simulink model "ASM_Traffic_MultiCore"  (R2026a)
settings: Solver=ode1  StartTime=SIM.tstart.v  StopTime=SIM.tend.v  FixedStep=SIM.StepSize.v
PostLoadFcn:
  | if any(exist('dsrtsu_mdlpostloadfcn', 'file') ~= 0), dsrtsu_mdlpostloadfcn('Execute', bdroot); end
  | try, asm_mdl_postloadfcn(bdroot, 'UpdateModel', 3600); catch, disp(lasterr); end,
InitFcn:
  | , if any(exist('rtifpga_mdlclblib', 'file') ~= 0), rtifpga_mdlclblib('Init', bdroot); end,
  | , if any(exist('dsmpb_private', 'file') ~= 0), dsmpb_private('dsmpb_mdlclblib', 'Init', bdroot); end,
model workspace (MAT data in the model file):
  asmReferencePath = [0 0.01 0.02 0.03 0.04 0.05 0.06 0.07 0.08 0.09 0.1 0.11 ... (350007 elements, 50001x7)]
  roadBounds : Simulink.Parameter (value not decoded)
  safetyAxes : Simulink.Parameter (value not decoded)
undefined symbols (not defined in the file): _to_, a0b2, ASM_BrakeHydraulics_DemoSystems, ASM_VehicleDynamics_DemoSystems, b98103fe8ad365046cd0, BrakeCircuit, controllerConfig, CPT, Crankshaft, DiscIntNeverNeededParam, dsmsi, FinalDriveAssembly, MDL, ModeSignals, mu, Pos_BrakePedal_Maneuver, rad, RefSignals, roadFamilyData, roadFamilyId, s_to_rpm, SIM, SoftECU, Suspension, Tire, Transmission
libraries: ASM_Traffic_lib x135, simulink x98, ASM_Utils_lib x77, ASM_VehicleDynamics_lib x70, ASM_Environment_lib x22, dsmpblib x20, dsmsilib x15, MDLD_Utils_lib x10, ASM_BrakeHydraulics_lib x3, sl_discontinuities x2
(part 24 of 65)

== system ASM_Traffic_MultiCore/Engine/Control/UserInterface/DISP_Control ==
  In : Inport
  Bus Selector2 : BusSelector  OutputSignals=Torque_Intervention.Enable_Trq_Request_Fast[0|1],Torque_Intervention.Enable_Trq_Request_Extern1[0|1],Torque_Intervention.Enable_Trq_Request_Extern2[0|1],Torque_Intervention.Enable_Trq_Request_Extern3[0|1],Torque_Intervention.Trq_Request_Fast[Nm],Torque_Intervention.Trq_Request_Extern1[Nm],Torque_Intervention.Trq_Request_Extern2[Nm],Torque_Intervention.Trq_Request_Extern3[Nm],Torque_Intervention.Pos_AccPedal_Request_Driver[%],Torque_Intervention.Pos_AccPedal_Request[%],EngineOperation.State_Engine[0|1|2|3|4],EngineOperation.Sw_Starter[0Off|1On]
  Enable_Trq_Request_Extern1[0|1] : Subsystem
      mask Display: disp('')
  Enable_Trq_Request_Extern2[0|1] : Subsystem
      mask Display: disp('')
  Enable_Trq_Request_Extern3[0|1] : Subsystem
      mask Display: disp('')
  Enable_Trq_Request_Fast[0|1] : Subsystem
      mask Display: disp('')
  Mux1 : Mux
  Mux2 : Mux  Inputs=2
  Mux3 : Mux
  Mux4 : Mux  Inputs=2
  Pos_AccPedal_Request[%] : Subsystem
      mask Display: disp('')
  Pos_AccPedal_Request_Driver[%] : Subsystem
      mask Display: disp('')
  SoftECU_Engine : Scope  NumInputPorts=4
      settings: TimeSpan=5  ActiveDisplayYMinimum=-42.03413  ActiveDisplayYMaximum=378.30719  DataLoggingMaxPoints=20000  DataLoggingDecimation=10
  State_Engine[0|1|2|3|4] : Subsystem
      mask Display: disp('')
  Sw_Starter[0|1] : Subsystem
      mask Display: disp('')
  Trq_Request_Extern1[Nm] : Subsystem
      mask Display: disp('')
  Trq_Request_Extern2[Nm] : Subsystem
      mask Display: disp('')
  Trq_Request_Extern3[Nm] : Subsystem
      mask Display: disp('')
  Trq_Request_Fast[Nm] : Subsystem
      mask Display: disp('')
  wires:
  In/1 -> Bus Selector2/1
  Bus Selector2/1 -> Enable_Trq_Request_Fast[0|1]/1(In1)  "<Enable_Trq_Request_Fast[0|1]>"
  Bus Selector2/2 -> Enable_Trq_Request_Extern1[0|1]/1(In1)  "<Enable_Trq_Request_Extern1[0|1]>"
  Bus Selector2/3 -> Enable_Trq_Request_Extern2[0|1]/1(In1)  "<Enable_Trq_Request_Extern2[0|1]>"
  Bus Selector2/4 -> Enable_Trq_Request_Extern3[0|1]/1(In1)  "<Enable_Trq_Request_Extern3[0|1]>"
  Bus Selector2/5 -> Trq_Request_Fast[Nm]/1(In1)  "<Trq_Request_Fast[Nm]>"
  Bus Selector2/6 -> Trq_Request_Extern1[Nm]/1(In1)  "<Trq_Request_Extern1[Nm]>"
  Bus Selector2/7 -> Trq_Request_Extern2[Nm]/1(In1)  "<Trq_Request_Extern2[Nm]>"
  Bus Selector2/8 -> Trq_Request_Extern3[Nm]/1(In1)  "<Trq_Request_Extern3[Nm]>"
  Bus Selector2/9 -> Pos_AccPedal_Request_Driver[%]/1(In1)  "<Pos_AccPedal_Request_Driver[%]>"
  Bus Selector2/10 -> Pos_AccPedal_Request[%]/1(In1)  "<Pos_AccPedal_Request[%]>"
  Bus Selector2/11 -> State_Engine[0|1|2|3|4]/1(In1)  "<State_Engine[0|1|2|3|4]>"
  Bus Selector2/12 -> Sw_Starter[0|1]/1(In1)  "<Sw_Starter[0Off|1On]>"
  Enable_Trq_Request_Fast[0|1]/1(Out1) -> Mux3/1
  Enable_Trq_Request_Extern1[0|1]/1(Out1) -> Mux3/2
  Enable_Trq_Request_Extern2[0|1]/1(Out1) -> Mux3/3
  Enable_Trq_Request_Extern3[0|1]/1(Out1) -> Mux3/4
  Trq_Request_Fast[Nm]/1(Out1) -> Mux1/1
  Trq_Request_Extern1[Nm]/1(Out1) -> Mux1/2
  Trq_Request_Extern2[Nm]/1(Out1) -> Mux1/3
  Trq_Request_Extern3[Nm]/1(Out1) -> Mux1/4
  Pos_AccPedal_Request_Driver[%]/1(Out1) -> Mux2/1
  Pos_AccPedal_Request[%]/1(Out1) -> Mux2/2
  Mux2/1 -> SoftECU_Engine/3
  State_Engine[0|1|2|3|4]/1(Out1) -> Mux4/1
  Sw_Starter[0|1]/1(Out1) -> Mux4/2
  Mux3/1 -> SoftECU_Engine/1
  Mux1/1 -> SoftECU_Engine/2
  Mux4/1 -> SoftECU_Engine/4

== system ASM_Traffic_MultiCore/Engine/Control/UserInterface/PAR_Control ==
  Termination : Constant  Value=0
  Out : Outport  VectorParamsAs1DForOutWhenUnconnected=off
  wires:
  Termination/1 -> Out/1

== system ASM_Traffic_MultiCore/Engine/Interface_In/ModelSignals/Enable_Trq_Decrease_Fast_ESP[0|1]_ ==
  In1 : Inport
  Gain : Gain  SaturateOnIntegerOverflow=on  OutDataTypeStr=Inherit: Same as input  ParamDataTypeStr=Inherit: Same as input
  Out1 : Outport  VectorParamsAs1DForOutWhenUnconnected=off
  wires:
  In1/1 -> Gain/1
  Gain/1 -> Out1/1

== system ASM_Traffic_MultiCore/Engine/Interface_In/ModelSignals/Enable_Trq_Increase_Fast_ESP[0|1]_ ==
  In1 : Inport
  Gain : Gain  SaturateOnIntegerOverflow=on  OutDataTypeStr=Inherit: Same as input  ParamDataTypeStr=Inherit: Same as input
  Out1 : Outport  VectorParamsAs1DForOutWhenUnconnected=off
  wires:
  In1/1 -> Gain/1
  Gain/1 -> Out1/1

== system ASM_Traffic_MultiCore/Engine/Interface_In/ModelSignals/Enable_Trq_Request_Extern1[0|1]_ ==
  In1 : Inport
  Gain : Gain  SaturateOnIntegerOverflow=on  OutDataTypeStr=Inherit: Same as input  ParamDataTypeStr=Inherit: Same as input
  Out1 : Outport  VectorParamsAs1DForOutWhenUnconnected=off
  wires:
  In1/1 -> Gain/1
  Gain/1 -> Out1/1

== system ASM_Traffic_MultiCore/Engine/Interface_In/ModelSignals/Enable_Trq_Request_Extern2[0|1]_ ==
  In1 : Inport
  Gain : Gain  SaturateOnIntegerOverflow=on  OutDataTypeStr=Inherit: Same as input  ParamDataTypeStr=Inherit: Same as input
  Out1 : Outport  VectorParamsAs1DForOutWhenUnconnected=off
  wires:
  In1/1 -> Gain/1
  Gain/1 -> Out1/1

== system ASM_Traffic_MultiCore/Engine/Interface_In/ModelSignals/Enable_n_Engine_Idle_Request[0|1]_ ==
  In1 : Inport
  Gain : Gain  SaturateOnIntegerOverflow=on  OutDataTypeStr=Inherit: Same as input  ParamDataTypeStr=Inherit: Same as input
  Out1 : Outport  VectorParamsAs1DForOutWhenUnconnected=off
  wires:
  Gain/1 -> Out1/1
  In1/1 -> Gain/1

== system ASM_Traffic_MultiCore/Engine/Interface_In/ModelSignals/Factor_Trq_Engine_Red[%]_ ==
  In1 : Inport
  Gain : Gain  SaturateOnIntegerOverflow=on  OutDataTypeStr=Inherit: Same as input  ParamDataTypeStr=Inherit: Same as input
  Out1 : Outport  VectorParamsAs1DForOutWhenUnconnected=off
  wires:
  In1/1 -> Gain/1
  Gain/1 -> Out1/1

== system ASM_Traffic_MultiCore/Engine/Interface_In/ModelSignals/Mode_StartButtonState[1Stim|2SoftECU]_ ==
  In1 : Inport
  Gain : Gain  SaturateOnIntegerOverflow=on  OutDataTypeStr=Inherit: Same as input  ParamDataTypeStr=Inherit: Same as input
  Out1 : Outport  VectorParamsAs1DForOutWhenUnconnected=off
  wires:
  In1/1 -> Gain/1
  Gain/1 -> Out1/1

== system ASM_Traffic_MultiCore/Engine/Interface_In/ModelSignals/Pos_AccPedal_Driver[%]_ ==
  In1 : Inport
  Gain : Gain  SaturateOnIntegerOverflow=on  OutDataTypeStr=Inherit: Same as input  ParamDataTypeStr=Inherit: Same as input
  Out1 : Outport  VectorParamsAs1DForOutWhenUnconnected=off
  wires:
  In1/1 -> Gain/1
  Gain/1 -> Out1/1

== system ASM_Traffic_MultiCore/Engine/Interface_In/ModelSignals/Reset_States[0|1]_ ==
  In1 : Inport
  Gain : Gain  SaturateOnIntegerOverflow=on  OutDataTypeStr=Inherit: Same as input  ParamDataTypeStr=Inherit: Same as input
  Out1 : Outport  VectorParamsAs1DForOutWhenUnconnected=off
  wires:
  In1/1 -> Gain/1
  Gain/1 -> Out1/1

== system ASM_Traffic_MultiCore/Engine/Interface_In/ModelSignals/State_StartButton[-1|0|1|2]_ ==
  In1 : Inport
  Gain : Gain  SaturateOnIntegerOverflow=on  OutDataTypeStr=Inherit: Same as input  ParamDataTypeStr=Inherit: Same as input
  Out1 : Outport  VectorParamsAs1DForOutWhenUnconnected=off
  wires:
  Gain/1 -> Out1/1
  In1/1 -> Gain/1

== system ASM_Traffic_MultiCore/Engine/Interface_In/ModelSignals/Sw_CrankShaft_Reset[0Disabled|1Enabled]_ ==
  In1 : Inport
  Gain : Gain  SaturateOnIntegerOverflow=on  OutDataTypeStr=Inherit: Same as input  ParamDataTypeStr=Inherit: Same as input
  Out1 : Outport  VectorParamsAs1DForOutWhenUnconnected=off
  wires:
  In1/1 -> Gain/1
  Gain/1 -> Out1/1

== system ASM_Traffic_MultiCore/Engine/Interface_In/ModelSignals/Sw_Ignition[0Off|1On]_ ==
  In1 : Inport
  Gain : Gain  SaturateOnIntegerOverflow=on  OutDataTypeStr=Inherit: Same as input  ParamDataTypeStr=Inherit: Same as input
  Out1 : Outport  VectorParamsAs1DForOutWhenUnconnected=off
  wires:
  In1/1 -> Gain/1
  Gain/1 -> Out1/1

== system ASM_Traffic_MultiCore/Engine/Interface_In/ModelSignals/Sw_ModelDeskPlottingInterface[0Disabled|1Enabled]_ ==
  In1 : Inport
  Gain : Gain
  Out1 : Outport
  wires:
  Gain/1 -> Out1/1
  In1/1 -> Gain/1

== system ASM_Traffic_MultiCore/Engine/Interface_In/ModelSignals/Sw_ModelPortBlocks[0Disabled|1Enabled]_ ==
  In1 : Inport
  Gain : Gain
  Out1 : Outport
  wires:
  Gain/1 -> Out1/1
  In1/1 -> Gain/1

== system ASM_Traffic_MultiCore/Engine/Interface_In/ModelSignals/Sw_StarterReq[0Off|1On]_ ==
  In1 : Inport
  Gain : Gain  SaturateOnIntegerOverflow=on  OutDataTypeStr=Inherit: Same as input  ParamDataTypeStr=Inherit: Same as input
  Out1 : Outport  VectorParamsAs1DForOutWhenUnconnected=off
  wires:
  In1/1 -> Gain/1
  Gain/1 -> Out1/1

== system ASM_Traffic_MultiCore/Engine/Interface_In/ModelSignals/Trq_Decrease_Request_Fast_ESP[Nm]_ ==
  In1 : Inport
  Gain : Gain  SaturateOnIntegerOverflow=on  OutDataTypeStr=Inherit: Same as input  ParamDataTypeStr=Inherit: Same as input
  Out1 : Outport  VectorParamsAs1DForOutWhenUnconnected=off
  wires:
  In1/1 -> Gain/1
  Gain/1 -> Out1/1

== system ASM_Traffic_MultiCore/Engine/Interface_In/ModelSignals/Trq_Increase_Request_Fast_ESP[Nm]_ ==
  In1 : Inport
  Gain : Gain  SaturateOnIntegerOverflow=on  OutDataTypeStr=Inherit: Same as input  ParamDataTypeStr=Inherit: Same as input
  Out1 : Outport  VectorParamsAs1DForOutWhenUnconnected=off
  wires:
  In1/1 -> Gain/1
  Gain/1 -> Out1/1

== system ASM_Traffic_MultiCore/Engine/Interface_In/ModelSignals/Trq_Request_Extern1[Nm]_ ==
  In1 : Inport
  Gain : Gain  SaturateOnIntegerOverflow=on  OutDataTypeStr=Inherit: Same as input  ParamDataTypeStr=Inherit: Same as input
  Out1 : Outport  VectorParamsAs1DForOutWhenUnconnected=off
  wires:
  In1/1 -> Gain/1
  Gain/1 -> Out1/1

== system ASM_Traffic_MultiCore/Engine/Interface_In/ModelSignals/Trq_Request_Extern2[Nm]_ ==
  In1 : Inport
  Gain : Gain  SaturateOnIntegerOverflow=on  OutDataTypeStr=Inherit: Same as input  ParamDataTypeStr=Inherit: Same as input
  Out1 : Outport  VectorParamsAs1DForOutWhenUnconnected=off
  wires:
  In1/1 -> Gain/1
  Gain/1 -> Out1/1

== system ASM_Traffic_MultiCore/Engine/Interface_In/ModelSignals/Trq_Request_ICE[Nm]_ ==
  In1 : Inport
  Gain : Gain  SaturateOnIntegerOverflow=on  OutDataTypeStr=Inherit: Same as input  ParamDataTypeStr=Inherit: Same as input
  Out1 : Outport  VectorParamsAs1DForOutWhenUnconnected=off
  wires:
  In1/1 -> Gain/1
  Gain/1 -> Out1/1

== system ASM_Traffic_MultiCore/Engine/Interface_In/ModelSignals/Vehicle_Topology[-2|-1|0|2]_ ==
  In1 : Inport
  Gain : Gain  SaturateOnIntegerOverflow=on  OutDataTypeStr=Inherit: Same as input  ParamDataTypeStr=Inherit: Same as input
  Out1 : Outport  VectorParamsAs1DForOutWhenUnconnected=off
  wires:
  In1/1 -> Gain/1
  Gain/1 -> Out1/1

== system ASM_Traffic_MultiCore/Engine/Interface_In/ModelSignals/n_Engine[rpm]_ ==
  In1 : Inport
  Gain : Gain  SaturateOnIntegerOverflow=on  OutDataTypeStr=Inherit: Same as input  ParamDataTypeStr=Inherit: Same as input
  Out1 : Outport  VectorParamsAs1DForOutWhenUnconnected=off
  wires:
  In1/1 -> Gain/1
  Gain/1 -> Out1/1

== system ASM_Traffic_MultiCore/Engine/Interface_In/ModelSignals/n_Engine_Idle_Request[rpm]_ ==
  In1 : Inport
  Gain : Gain  SaturateOnIntegerOverflow=on  OutDataTypeStr=Inherit: Same as input  ParamDataTypeStr=Inherit: Same as input
  Out1 : Outport  VectorParamsAs1DForOutWhenUnconnected=off
  wires:
  In1/1 -> Gain/1
  Gain/1 -> Out1/1

== system ASM_Traffic_MultiCore/Engine/Interface_In/ModelSignals/v_x_Vehicle[km|h]_ ==
  In1 : Inport
  Gain : Gain  SaturateOnIntegerOverflow=on  OutDataTypeStr=Inherit: Same as input  ParamDataTypeStr=Inherit: Same as input
  Out1 : Outport  VectorParamsAs1DForOutWhenUnconnected=off
  wires:
  In1/1 -> Gain/1
  Gain/1 -> Out1/1

== system ASM_Traffic_MultiCore/Engine/Interface_Out/Control_ModelSignals/CrankAngle_Cyl[aTDC]_ ==
  In1 : Inport
  DummyGain : Gain  SaturateOnIntegerOverflow=on  OutDataTypeStr=Inherit: Same as input  ParamDataTypeStr=Inherit: Same as input
  Out1 : Outport  VectorParamsAs1DForOutWhenUnconnected=off
  wires:
  DummyGain/1 -> Out1/1
  In1/1 -> DummyGain/1

== system ASM_Traffic_MultiCore/Engine/Interface_Out/Control_ModelSignals/Enable_Trq_Shift_Request[0|1]_ ==
  In1 : Inport
  Gain : Gain  SaturateOnIntegerOverflow=on  OutDataTypeStr=Inherit: Same as input  ParamDataTypeStr=Inherit: Same as input
  Out1 : Outport  VectorParamsAs1DForOutWhenUnconnected=off
  wires:
  Gain/1 -> Out1/1
  In1/1 -> Gain/1

== system ASM_Traffic_MultiCore/Engine/Interface_Out/Control_ModelSignals/EngOP_Num[]_ ==
  In1 : Inport
  DummyGain : Gain  SaturateOnIntegerOverflow=on  OutDataTypeStr=Inherit: Same as input  ParamDataTypeStr=Inherit: Same as input
  Out1 : Outport  VectorParamsAs1DForOutWhenUnconnected=off
  wires:
  In1/1 -> DummyGain/1
  DummyGain/1 -> Out1/1

== system ASM_Traffic_MultiCore/Engine/Interface_Out/Control_ModelSignals/Pos_AccPedal_Meas[%]_ ==
  In1 : Inport
  DummyGain : Gain  SaturateOnIntegerOverflow=on  OutDataTypeStr=Inherit: Same as input  ParamDataTypeStr=Inherit: Same as input
  Out1 : Outport  VectorParamsAs1DForOutWhenUnconnected=off
  wires:
  DummyGain/1 -> Out1/1
  In1/1 -> DummyGain/1

== system ASM_Traffic_MultiCore/Engine/Interface_Out/Control_ModelSignals/State_ICEngine[0|1|2|3|4]_ ==
  In1 : Inport
  Gain : Gain  SaturateOnIntegerOverflow=on  OutDataTypeStr=Inherit: Same as input  ParamDataTypeStr=Inherit: Same as input
  Out1 : Outport  VectorParamsAs1DForOutWhenUnconnected=off
  wires:
  In1/1 -> Gain/1
  Gain/1 -> Out1/1

== system ASM_Traffic_MultiCore/Engine/Interface_Out/Control_ModelSignals/State_StartStop[1Off|2NotReady|3Ready|4EngStopped]_ ==
  In1 : Inport
  Gain : Gain  SaturateOnIntegerOverflow=on  OutDataTypeStr=Inherit: Same as input  ParamDataTypeStr=Inherit: Same as input
  Out1 : Outport  VectorParamsAs1DForOutWhenUnconnected=off
  wires:
  In1/1 -> Gain/1
  Gain/1 -> Out1/1

== system ASM_Traffic_MultiCore/Engine/Interface_Out/Control_ModelSignals/Sw_Replace_Env[0|1]_ ==
  In1 : Inport
  DummyGain : Gain  SaturateOnIntegerOverflow=on  OutDataTypeStr=Inherit: Same as input  ParamDataTypeStr=Inherit: Same as input
  Out1 : Outport  VectorParamsAs1DForOutWhenUnconnected=off
  wires:
  DummyGain/1 -> Out1/1
  In1/1 -> DummyGain/1

== system ASM_Traffic_MultiCore/Engine/Interface_Out/Control_ModelSignals/Sw_Starter[0Off|1On]_ ==
  In1 : Inport
  Gain : Gain  SaturateOnIntegerOverflow=on  OutDataTypeStr=Inherit: Same as input  ParamDataTypeStr=Inherit: Same as input
  Out1 : Outport  VectorParamsAs1DForOutWhenUnconnected=off
  wires:
  In1/1 -> Gain/1
  Gain/1 -> Out1/1

== system ASM_Traffic_MultiCore/Engine/Interface_Out/Control_ModelSignals/T_Ambient[degC]_ ==
  In1 : Inport
  DummyGain : Gain  SaturateOnIntegerOverflow=on  OutDataTypeStr=Inherit: Same as input  ParamDataTypeStr=Inherit: Same as input
  Out1 : Outport  VectorParamsAs1DForOutWhenUnconnected=off
  wires:
  DummyGain/1 -> Out1/1
  In1/1 -> DummyGain/1

== system ASM_Traffic_MultiCore/Engine/Interface_Out/Control_ModelSignals/Trq_MeanEff_Engine_Meas[Nm]_ ==
  In1 : Inport
  DummyGain : Gain  SaturateOnIntegerOverflow=on  OutDataTypeStr=Inherit: Same as input  ParamDataTypeStr=Inherit: Same as input
  Out1 : Outport  VectorParamsAs1DForOutWhenUnconnected=off
  wires:
  DummyGain/1 -> Out1/1
  In1/1 -> DummyGain/1

== system ASM_Traffic_MultiCore/Engine/Interface_Out/Control_ModelSignals/Trq_Shift_Request[Nm]_ ==
  In1 : Inport
  Gain : Gain  SaturateOnIntegerOverflow=on  OutDataTypeStr=Inherit: Same as input  ParamDataTypeStr=Inherit: Same as input
  Out1 : Outport  VectorParamsAs1DForOutWhenUnconnected=off
  wires:
  In1/1 -> Gain/1
  Gain/1 -> Out1/1

== system ASM_Traffic_MultiCore/Engine/Interface_Out/Control_ModelSignals/n_Engine_Idle_Set[rpm]_ ==
  In1 : Inport
  Gain : Gain  SaturateOnIntegerOverflow=on  OutDataTypeStr=Inherit: Same as input  ParamDataTypeStr=Inherit: Same as input
  Out1 : Outport  VectorParamsAs1DForOutWhenUnconnected=off
  wires:
  In1/1 -> Gain/1
  Gain/1 -> Out1/1

== system ASM_Traffic_MultiCore/Engine/Interface_Out/Control_ModelSignals/n_Engine_Meas[rpm]_ ==
  In1 : Inport
  DummyGain : Gain  SaturateOnIntegerOverflow=on  OutDataTypeStr=Inherit: Same as input  ParamDataTypeStr=Inherit: Same as input
  Out1 : Outport  VectorParamsAs1DForOutWhenUnconnected=off
  wires:
  In1/1 -> DummyGain/1
  DummyGain/1 -> Out1/1

== system ASM_Traffic_MultiCore/Engine/Interface_Out/Control_ModelSignals/p_Ambient[Pa]_ ==
  In1 : Inport
  DummyGain : Gain  SaturateOnIntegerOverflow=on  OutDataTypeStr=Inherit: Same as input  ParamDataTypeStr=Inherit: Same as input
  Out1 : Outport  VectorParamsAs1DForOutWhenUnconnected=off
  wires:
  In1/1 -> DummyGain/1
  DummyGain/1 -> Out1/1

== system ASM_Traffic_MultiCore/Engine/Interface_Out/Plant_ModelSignals/T_Coolant_ICE[degC]_ ==
  In1 : Inport
  Gain : Gain  SaturateOnIntegerOverflow=on  OutDataTypeStr=Inherit: Same as input  ParamDataTypeStr=Inherit: Same as input
  Out1 : Outport  VectorParamsAs1DForOutWhenUnconnected=off
  wires:
  Gain/1 -> Out1/1
  In1/1 -> Gain/1

== system ASM_Traffic_MultiCore/Engine/Interface_Out/Plant_ModelSignals/Trq_Fric_Engine[Nm]_ ==
  In1 : Inport
  Gain : Gain  SaturateOnIntegerOverflow=on  OutDataTypeStr=Inherit: Same as input  ParamDataTypeStr=Inherit: Same as input
  Out1 : Outport  VectorParamsAs1DForOutWhenUnconnected=off
  wires:
  In1/1 -> Gain/1
  Gain/1 -> Out1/1

== system ASM_Traffic_MultiCore/Engine/Interface_Out/Plant_ModelSignals/Trq_MeanEff_Engine[Nm]_ ==
  In1 : Inport
  Gain : Gain  SaturateOnIntegerOverflow=on  OutDataTypeStr=Inherit: Same as input  ParamDataTypeStr=Inherit: Same as input
  Out1 : Outport  VectorParamsAs1DForOutWhenUnconnected=off
  wires:
  In1/1 -> Gain/1
  Gain/1 -> Out1/1

== system ASM_Traffic_MultiCore/Engine/Interface_Out/Plant_ModelSignals/Type_Engine[0Unkown|1Other|2Otto|3Diesel|4Electric]_ ==
  In1 : Inport
  DummyGain : Gain  SaturateOnIntegerOverflow=on  OutDataTypeStr=Inherit: Same as input  ParamDataTypeStr=Inherit: Same as input
  Out1 : Outport  VectorParamsAs1DForOutWhenUnconnected=off
  wires:
  In1/1 -> DummyGain/1
  DummyGain/1 -> Out1/1

== system ASM_Traffic_MultiCore/Engine/Plant/EngineBasic/ASMSignalCollector ==
  BusCreator : BusCreator  Inputs=2
  ASMSIgnalBus : Outport  VectorParamsAs1DForOutWhenUnconnected=off
  wires:
  [ASMBUS_FUEL_CONSUMPTION] -> BusCreator/2
  BusCreator/1 -> ASMSIgnalBus/1  "Plant"
  [ASMBUS_ENGINE] -> BusCreator/1

== system ASM_Traffic_MultiCore/Engine/Plant/UserInterface/ASMSignalBus_Plant ==
  In : Inport
  Terminator_1 : Terminator
  tag scope: ASMBUS_Engine_Plant=global
  wires:
  [ASMBUS_Engine_Plant] -> Terminator_1/1
  In/1 -> [ASMBUS_Engine_Plant]  "Plant"

== system ASM_Traffic_MultiCore/Engine/Plant/UserInterface/DISP_Plant ==
  note: Dummy blocks for ControlDesk layout.
      | Might be replaced when simulating virtual vehicles.
  Interface_In : Inport
  In : Inport  Port=2
  Bus Selector1 : BusSelector  OutputSignals=Engine.Trq_Eff_Engine[Nm],Engine.Trq_Fric_Engine[Nm],Engine.Trq_Ind_Engine[Nm]
  Bus Selector10 : BusSelector  OutputSignals=FuelConsumption.CO2_Emission.CO2_Emission[kg|h],FuelConsumption.CO2_Emission.CO2_Emission_Total[kg],FuelConsumption.Fuel_Consumption[l|h],FuelConsumption.Fuel_Consumption_Total[l],FuelConsumption.mdot_Fuel[g|h],FuelConsumption.b_e[g|kWh],FuelConsumption.Efficiency.eta_Eff_Engine[0_1],FuelConsumption.Efficiency.eta_Ind_Engine[0_1],FuelConsumption.Efficiency.eta_Mechanical_Engine[0_1]
  Bus Selector2 : BusSelector  OutputSignals=ExternalModel.v_x_Vehicle[km|h]
  CO2_Emission[kg|100km] : Subsystem
      mask Display: disp('')
  CO2_Emission[kg|100km]_ : Subsystem
  CO2_Emission[kg|h] : Subsystem
      mask Display: disp('')
  CO2_Emission_Total[kg] : Subsystem
      mask Display: disp('')
  CarbonEmission : Scope  NumInputPorts=3
      settings: TimeSpan=5  ActiveDisplayYMinimum=98.25  ActiveDisplayYMaximum=102.25  DataLoggingMaxPoints=20000  DataLoggingDecimation=10  DataLoggingVariableName=ScopeData3
  Efficiency : Scope  NumInputPorts=3
      settings: TimeSpan=5  ActiveDisplayYMinimum=-0.1  ActiveDisplayYMaximum=0.6  DataLoggingMaxPoints=20000  DataLoggingDecimation=10  DataLoggingVariableName=ScopeData4
  Engine : Scope  NumInputPorts=3
      settings: TimeSpan=5  ActiveDisplayYMinimum=-20  ActiveDisplayYMaximum=110  DataLoggingMaxPoints=20000  DataLoggingDecimation=10  DataLoggingVariableName=ScopeData5
  FuelConsumption : Scope  NumInputPorts=5
      settings: TimeSpan=5  ActiveDisplayYMinimum=2100  ActiveDisplayYMaximum=2300  DataLoggingMaxPoints=20000  DataLoggingDecimation=10  DataLoggingVariableName=ScopeData6
  FuelTank : Constant  Value=0.5
  FuelTank[0|1] : Subsystem
      mask Display: disp('')
  Fuel_Consumption[L|100km] : Subsystem
      mask Display: disp('')
  Fuel_Consumption[L|100km]_ : Subsystem
  Fuel_Consumption[l|h] : Subsystem
      mask Display: disp('')
  Fuel_Consumption_Total[l] : Subsystem
      mask Display: disp('')
  T_Water : Constant
  T_Water[degC] : Subsystem
      mask Display: disp('')
  Terminator : Terminator
  Terminator2 : Terminator
  Trq_Eff_Engine[Nm] : Subsystem
      mask Display: disp('')
  Trq_Fric_Engine[Nm] : Subsystem
      mask Display: disp('')
  Trq_Ind_Engine[Nm] : Subsystem
      mask Display: disp('')
  b_e[g|kWh] : Subsystem
      mask Display: disp('')
  eta_Eff_Engine[0_1] : Subsystem
      mask Display: disp('')
  eta_Ind_Engine[0_1] : Subsystem
      mask Display: disp('')
  eta_Mechanical_Engine[0_1] : Subsystem
      mask Display: disp('')
  mdot_Fuel[g|h] : Subsystem
      mask Display: disp('')
  wires:
  Bus Selector2/1 -> CO2_Emission[kg|100km]_/1(v_Vehicle[km|h]), Fuel_Consumption[L|100km]_/1(v_Vehicle[km|h])  "<v_x_Vehicle[km|h]>"
  Interface_In/1 -> Bus Selector2/1
  Bus Selector10/4 -> Fuel_Consumption_Total[l]/1(In1)  "<Fuel_Consumption_Total[l]>"
  T_Water[degC]/1(Out1) -> Terminator2/1
  FuelTank/1 -> FuelTank[0|1]/1(In1)
  Fuel_Consumption[L|100km]/1(Out1) -> FuelConsumption/1  "Fuel_Conumption[l|100km]"
  T_Water/1 -> T_Water[degC]/1(In1)
  FuelTank[0|1]/1(Out1) -> Terminator/1
  Trq_Ind_Engine[Nm]/1(Out1) -> Engine/3  "Trq_Ind_Engine[Nm]"
  Bus Selector1/1 -> Trq_Eff_Engine[Nm]/1(In1)  "<Trq_Eff_Engine[Nm]>"
  Fuel_Consumption[L|100km]_/1(Fuel_Consumption[L|100km]) -> Fuel_Consumption[L|100km]/1(In1)
  Bus Selector1/3 -> Trq_Ind_Engine[Nm]/1(In1)  "<Trq_Ind_Engine[Nm]>"
  Trq_Fric_Engine[Nm]/1(Out1) -> Engine/2  "Trq_Fric_Engine[Nm]"
  CO2_Emission_Total[kg]/1(Out1) -> CarbonEmission/3  "CO2_Emission_Total[kg]"
  Bus Selector10/3 -> Fuel_Consumption[l|h]/1(In1), Fuel_Consumption[L|100km]_/2(Fuel_Consumption[l|h])  "<Fuel_Consumption[l|h]>"
  Bus Selector1/2 -> Trq_Fric_Engine[Nm]/1(In1)  "<Trq_Fric_Engine[Nm]>"
  CO2_Emission[kg|100km]_/1(CO2_Emission[kg|100km]) -> CO2_Emission[kg|100km]/1(In1)
  eta_Eff_Engine[0_1]/1(Out1) -> Efficiency/1  "eta_Eff_Engine[0_1]"
  Bus Selector10/5 -> mdot_Fuel[g|h]/1(In1)  "<mdot_Fuel[g|h]>"
  Bus Selector10/1 -> CO2_Emission[kg|h]/1(In1), CO2_Emission[kg|100km]_/2(CO2_Emission[kg|h])  "<CO2_Emission[kg|h]>"
  Bus Selector10/6 -> b_e[g|kWh]/1(In1)  "<b_e[g|kWh]>"
  Bus Selector10/2 -> CO2_Emission_Total[kg]/1(In1)  "<CO2_Emission_Total[kg]>"
  Trq_Eff_Engine[Nm]/1(Out1) -> Engine/1  "Trq_Eff_Engine[Nm]"
  CO2_Emission[kg|h]/1(Out1) -> CarbonEmission/2  "CO2_Emission[kg|h]"
  Bus Selector10/7 -> eta_Eff_Engine[0_1]/1(In1)  "<eta_Eff_Engine[0_1]>"
  Fuel_Consumption_Total[l]/1(Out1) -> FuelConsumption/3  "Fuel_Consumption_Total[l]"
  Bus Selector10/9 -> eta_Mechanical_Engine[0_1]/1(In1)  "<eta_Mechanical_Engine[0_1]>"
  In/1 -> Bus Selector1/1, Bus Selector10/1
  Fuel_Consumption[l|h]/1(Out1) -> FuelConsumption/2  "Fuel_Consumption[l|h]"
  eta_Mechanical_Engine[0_1]/1(Out1) -> Efficiency/3  "eta_Mechanical_Engine[0_1]"
  Bus Selector10/8 -> eta_Ind_Engine[0_1]/1(In1)  "<eta_Ind_Engine[0_1]>"
  eta_Ind_Engine[0_1]/1(Out1) -> Efficiency/2  "eta_Ind_Engine[0_1]"
  CO2_Emission[kg|100km]/1(Out1) -> CarbonEmission/1  "CO2_Emission[kg|100km]"
  b_e[g|kWh]/1(Out1) -> FuelConsumption/5  "b_e[g|kWh]"
  mdot_Fuel[g|h]/1(Out1) -> FuelConsumption/4  "mdot_Fuel[g|h]"

== system ASM_Traffic_MultiCore/Engine/Plant/UserInterface/PAR_Plant ==
  Termination : Constant  Value=0
  Out : Outport  VectorParamsAs1DForOutWhenUnconnected=off
  wires:
  Termination/1 -> Out/1

== system ASM_Traffic_MultiCore/Engine/SignalInterface/ASMSignalInterface/signal_structure ==
  ASMSignalBus : Inport
  BusSelector_1 : BusSelector  OutputSignals=Control,Plant
  CO2_Emission : BusSelector  OutputSignals=CO2_Emission[kg|h],CO2_Emission_Total[kg]
  ContentID : Constant  Value=278498219
  Control : BusSelector  OutputSignals=ESP_Fast_Torque_Set,Shift_Torque_Set,Torque_Intervention,IdleSpeedControl,EngineOperation
  DataTypeConversion_2 : DataTypeConversion  OutDataTypeStr=double
  ESP_Fast_Torque_Set : BusSelector  OutputSignals=Sw_Engine_Dynamics_Fast[0|1],Enable_Trq_Request_Fast[0|1],Trq_Request_Fast[Nm]
  Efficiency : BusSelector  OutputSignals=eta_Eff_Engine[0_1],eta_Ind_Engine[0_1],eta_Mechanical_Engine[0_1]
  Engine : BusSelector  OutputSignals=TimeConst_Engine_Dynamics[s],Trq_Eff_Engine[Nm],Trq_Driver_Des[Nm],Trq_FullLoad_Engine[Nm],Trq_Fric_Engine[Nm],Trq_Ind_Engine[Nm],Trq_Driver_Ind_Des[Nm],Trq_Engine_Ind_Max[Nm]
  EngineOperation : BusSelector  OutputSignals=State_Engine[0|1|2|3|4],Sw_Starter[0Off|1On]
  FuelConsumption : BusSelector  OutputSignals=mdot_Fuel[g|h],b_e[g|kWh],Efficiency,CO2_Emission,Fuel_Consumption[l|h],Fuel_Consumption_Total[l]
  IdleSpeedControl : BusSelector  OutputSignals=n_Engine_Idle_Set[rpm],Pos_AccPedal_Ctrl[%]
  InfoBlock : Subsystem
      mask Display: fprintf('Structural changes of the signal bus require an update \nof the ''ASMSignalCollector'' block. \n\nTo start the update process double click the parent block.\n\n WARNING:\n During update this subsystem will be cleared completely')
  MDLD_DATA_CAPTURE : MDLD_Utils_lib/ModelDeskPlotInterface/DataCapture_Sfcn/MDLD_DATA_CAPTURE  inputPortWidth=41  measurementSignals=[0 0 0 0 0 0 0 0 0 0 0 0 0 0 0 0 0 0 0 0 0 0 0 0 0 0 0 0 0 0 0 0 0 0 0 0 0 0 0 0 0]  downsampling=1  samplingPeriod=SIM.StepSize.v  uuid=0  ASMProperties=struct('Name','mdld_data_capture','Version','1.0','Library','mdld_utils_lib')  startTriggerDelay=0  startTriggerLogic=0  startTriggerCount=0  startTriggerConditions=[0,0,0,0,0,0,0,0,0]  stopTriggerDelay=0  stopTriggerLogic=0  stopTriggerCount=0  stopTriggerConditions=[0,0,0,0,0,0,0,0,0]  ContentID_RefStruct=278498219
  Plant : BusSelector  OutputSignals=Engine,FuelConsumption
  Shift_Torque_Set : BusSelector  OutputSignals=Trq_Driver_Ind_Des[Nm],Trq_Ind_Set[Nm],Enable_Trq_Ind_Set[0|1]
  SignalFilter : Mux  Inputs=41
  SignalFilterGain : Gain
  Terminator : Terminator
  Torque_Intervention : BusSelector  OutputSignals=Pos_AccPedal_Request[%],Enable_Trq_Request_Fast[0|1],Enable_Trq_Request_Extern1[0|1],Enable_Trq_Request_Extern2[0|1],Enable_Trq_Request_Extern3[0|1],Trq_Request_Fast[Nm],Trq_Request_Extern1[Nm],Trq_Request_Extern2[Nm],Trq_Request_Extern3[Nm],Pos_AccPedal_Request_Fast[%],Pos_AccPedal_Request_Extern1[%],Pos_AccPedal_Request_Extern2[%],Pos_AccPedal_Request_Extern3[%],Pos_AccPedal_Request_Driver[%]
  wires:
  ASMSignalBus/1 -> BusSelector_1/1
  BusSelector_1/1 -> Control/1  "<Control>"
  Control/1 -> ESP_Fast_Torque_Set/1  "<ESP_Fast_Torque_Set>"
  Control/2 -> Shift_Torque_Set/1  "<Shift_Torque_Set>"
  Control/3 -> Torque_Intervention/1  "<Torque_Intervention>"
  Control/4 -> IdleSpeedControl/1  "<IdleSpeedControl>"
  Control/5 -> EngineOperation/1  "<EngineOperation>"
  BusSelector_1/2 -> Plant/1  "<Plant>"
  Plant/1 -> Engine/1  "<Engine>"
  Plant/2 -> FuelConsumption/1  "<FuelConsumption>"
  FuelConsumption/3 -> Efficiency/1  "<Efficiency>"
  FuelConsumption/4 -> CO2_Emission/1  "<CO2_Emission>"
  ContentID/1 -> Terminator/1
  ESP_Fast_Torque_Set/1 -> SignalFilter/1  "<Sw_Engine_Dynamics_Fast[0|1]>"
  ESP_Fast_Torque_Set/2 -> DataTypeConversion_2/1  "<Enable_Trq_Request_Fast[0|1]>"
  DataTypeConversion_2/1 -> SignalFilter/2
  ESP_Fast_Torque_Set/3 -> SignalFilter/3  "<Trq_Request_Fast[Nm]>"
  Shift_Torque_Set/1 -> SignalFilter/4  "<Trq_Driver_Ind_Des[Nm]>"
  Shift_Torque_Set/2 -> SignalFilter/5  "<Trq_Ind_Set[Nm]>"
  Shift_Torque_Set/3 -> SignalFilter/6  "<Enable_Trq_Ind_Set[0|1]>"
  Torque_Intervention/1 -> SignalFilter/7  "<Pos_AccPedal_Request[%]>"
  Torque_Intervention/2 -> SignalFilter/8  "<Enable_Trq_Request_Fast[0|1]>"
  Torque_Intervention/3 -> SignalFilter/9  "<Enable_Trq_Request_Extern1[0|1]>"
  Torque_Intervention/4 -> SignalFilter/10  "<Enable_Trq_Request_Extern2[0|1]>"
  Torque_Intervention/5 -> SignalFilter/11  "<Enable_Trq_Request_Extern3[0|1]>"
  Torque_Intervention/6 -> SignalFilter/12  "<Trq_Request_Fast[Nm]>"
  Torque_Intervention/7 -> SignalFilter/13  "<Trq_Request_Extern1[Nm]>"
  Torque_Intervention/8 -> SignalFilter/14  "<Trq_Request_Extern2[Nm]>"
  Torque_Intervention/9 -> SignalFilter/15  "<Trq_Request_Extern3[Nm]>"
  Torque_Intervention/10 -> SignalFilter/16  "<Pos_AccPedal_Request_Fast[%]>"
  Torque_Intervention/11 -> SignalFilter/17  "<Pos_AccPedal_Request_Extern1[%]>"
  Torque_Intervention/12 -> SignalFilter/18  "<Pos_AccPedal_Request_Extern2[%]>"
  Torque_Intervention/13 -> SignalFilter/19  "<Pos_AccPedal_Request_Extern3[%]>"
  Torque_Intervention/14 -> SignalFilter/20  "<Pos_AccPedal_Request_Driver[%]>"
  IdleSpeedControl/1 -> SignalFilter/21  "<n_Engine_Idle_Set[rpm]>"
  IdleSpeedControl/2 -> SignalFilter/22  "<Pos_AccPedal_Ctrl[%]>"
  EngineOperation/1 -> SignalFilter/23  "<State_Engine[0|1|2|3|4]>"
  EngineOperation/2 -> SignalFilter/24  "<Sw_Starter[0Off|1On]>"
  Engine/1 -> SignalFilter/25  "<TimeConst_Engine_Dynamics[s]>"
  Engine/2 -> SignalFilter/26  "<Trq_Eff_Engine[Nm]>"
  Engine/3 -> SignalFilter/27  "<Trq_Driver_Des[Nm]>"
  Engine/4 -> SignalFilter/28  "<Trq_FullLoad_Engine[Nm]>"
  Engine/5 -> SignalFilter/29  "<Trq_Fric_Engine[Nm]>"
  Engine/6 -> SignalFilter/30  "<Trq_Ind_Engine[Nm]>"
  Engine/7 -> SignalFilter/31  "<Trq_Driver_Ind_Des[Nm]>"
  Engine/8 -> SignalFilter/32  "<Trq_Engine_Ind_Max[Nm]>"
  FuelConsumption/1 -> SignalFilter/33  "<mdot_Fuel[g|h]>"
  FuelConsumption/2 -> SignalFilter/34  "<b_e[g|kWh]>"
  Efficiency/1 -> SignalFilter/35  "<eta_Eff_Engine[0_1]>"
  Efficiency/2 -> SignalFilter/36  "<eta_Ind_Engine[0_1]>"
  Efficiency/3 -> SignalFilter/37  "<eta_Mechanical_Engine[0_1]>"
  CO2_Emission/1 -> SignalFilter/38  "<CO2_Emission[kg|h]>"
  CO2_Emission/2 -> SignalFilter/39  "<CO2_Emission_Total[kg]>"
  FuelConsumption/5 -> SignalFilter/40  "<Fuel_Consumption[l|h]>"
  FuelConsumption/6 -> SignalFilter/41  "<Fuel_Consumption_Total[l]>"
  SignalFilter/1 -> SignalFilterGain/1
  SignalFilterGain/1 -> MDLD_DATA_CAPTURE/1

== system ASM_Traffic_MultiCore/Engine/SignalInterface/ExternalOutports/Select_Outport_Signals ==
  ASMSignalBus : Inport
  Bus Selector : BusSelector  OutputSignals=Plant.Engine,Plant.FuelConsumption
  Engine : Outport  VectorParamsAs1DForOutWhenUnconnected=off
  FuelConsumption : Outport  Port=2  VectorParamsAs1DForOutWhenUnconnected=off
  wires:
  ASMSignalBus/1 -> Bus Selector/1
  Bus Selector/1 -> Engine/1  "<Engine>"
  Bus Selector/2 -> FuelConsumption/1  "<FuelConsumption>"

== system ASM_Traffic_MultiCore/Environment/GroundTruth/PlantModel/Add_Time ==
  TimeSignal[s] : Inport
  Environmental_Conditions[] : Inport  Port=2
  Add : Sum
  Add1 : Sum
  Mux : Mux  Inputs=3
  Reset_Time : Subsystem
  Rounding Function : Rounding
  Saturation1 : Saturate  UpperLimit=inf  LowerLimit=0
  Selector : Selector  InputPortWidth=8  IndexOptions=Index vector (dialog)  Indices=7  OutputSizes=1
  Selector1 : Selector  InputPortWidth=8  IndexOptions=Index vector (dialog)  Indices=8  OutputSizes=1
  Selector2 : Selector  InputPortWidth=8  IndexOptions=Index vector (dialog)  Indices=(1:6)  OutputSizes=1
  EnvironmentConditions_Out[] : Outport  VectorParamsAs1DForOutWhenUnconnected=off
  wires:
  Mux/1 -> EnvironmentConditions_Out[]/1
  Selector2/1 -> Mux/1  "Environment_Signals_Rest[]"
  Reset_Time/1(Seconds_Out[s]) -> Mux/2  "Seconds_Since_Midnight[s]"
  Saturation1/1 -> Mux/3  "Unix_Timestamp[s]"
  Add/1 -> Saturation1/1
  Add1/1 -> Reset_Time/1(Seconds_In[s])
  Rounding Function/1 -> Add/1, Add1/1
  TimeSignal[s]/1 -> Rounding Function/1
  Selector1/1 -> Add/2  "Start_Unix_Timestamp[s]"
  Selector/1 -> Add1/2  "Start_Seconds_Since_Midnight[s]"
  Environmental_Conditions[]/1 -> Selector/1, Selector2/1, Selector1/1

== system ASM_Traffic_MultiCore/Environment/GroundTruth/PlantModel/AutomatedDrivingFunction[] ==
  In : Inport
  Bus Selector23 : BusSelector  OutputSignals=AutomatedDrivingFunction_ACC[],AutomatedDrivingFunction_AEB[],AutomatedDrivingFunction_FCW[],AutomatedDrivingFunction_4[]
  Bus_Selector_AutomatedDrivingFunction_4 : BusSelector  OutputSignals=Driver_Override_Active[0Off|1On],Driver_Override_Reason_Idx[],State_Idx[],Name_Idx[],Custom_Name_Idx[],Custom_State_Idx[],Key_1_Idx[],Value_1_Idx[],Key_2_Idx[],Value_2_Idx[]
  Bus_Selector_AutomatedDrivingFunction_ACC : BusSelector  OutputSignals=Driver_Override_Active[0Off|1On],Driver_Override_Reason_Idx[],State_Idx[],Name_Idx[],Custom_Name_Idx[],Custom_State_Idx[],Key_1_Idx[],Value_1_Idx[],Key_2_Idx[],Value_2_Idx[]
  Bus_Selector_AutomatedDrivingFunction_AEB : BusSelector  OutputSignals=Driver_Override_Reason_Idx[],Driver_Override_Reason_Idx[],State_Idx[],Name_Idx[],Custom_Name_Idx[],Custom_State_Idx[],Key_1_Idx[],Value_1_Idx[],Key_2_Idx[],Value_2_Idx[]
  Bus_Selector_AutomatedDrivingFunction_FCW : BusSelector  OutputSignals=Driver_Override_Active[0Off|1On],Driver_Override_Reason_Idx[],State_Idx[],Name_Idx[],Custom_Name_Idx[],Custom_State_Idx[],Key_1_Idx[],Value_1_Idx[],Key_2_Idx[],Value_2_Idx[]
  Mux4 : Mux
  Mux_AutomatedDrivingFunction_4 : Mux  Inputs=10
  Mux_AutomatedDrivingFunction_ACC : Mux  Inputs=10
  Mux_AutomatedDrivingFunction_AEB : Mux  Inputs=10
  Mux_AutomatedDrivingFunction_FCW : Mux  Inputs=10
  AutomatedDrivingFunction[] : Outport  VectorParamsAs1DForOutWhenUnconnected=off
  wires:
  In/1 -> Bus Selector23/1
  Bus Selector23/1 -> Bus_Selector_AutomatedDrivingFunction_ACC/1  "<AutomatedDrivingFunction_ACC[]>"
  Bus Selector23/2 -> Bus_Selector_AutomatedDrivingFunction_AEB/1  "<AutomatedDrivingFunction_AEB[]>"
  Bus Selector23/3 -> Bus_Selector_AutomatedDrivingFunction_FCW/1  "<AutomatedDrivingFunction_FCW[]>"
  Bus Selector23/4 -> Bus_Selector_AutomatedDrivingFunction_4/1  "<AutomatedDrivingFunction_4[]>"
  Bus_Selector_AutomatedDrivingFunction_ACC/1 -> Mux_AutomatedDrivingFunction_ACC/1  "<Driver_Override_Active[0Off|1On]>"
  Bus_Selector_AutomatedDrivingFunction_ACC/2 -> Mux_AutomatedDrivingFunction_ACC/2  "<Driver_Override_Reason_Idx[]>"
  Bus_Selector_AutomatedDrivingFunction_ACC/3 -> Mux_AutomatedDrivingFunction_ACC/3  "<State_Idx[]>"
  Bus_Selector_AutomatedDrivingFunction_ACC/4 -> Mux_AutomatedDrivingFunction_ACC/4  "<Name_Idx[]>"
  Bus_Selector_AutomatedDrivingFunction_ACC/5 -> Mux_AutomatedDrivingFunction_ACC/5  "<Custom_Name_Idx[]>"
  Bus_Selector_AutomatedDrivingFunction_ACC/6 -> Mux_AutomatedDrivingFunction_ACC/6  "<Custom_State_Idx[]>"
  Bus_Selector_AutomatedDrivingFunction_ACC/7 -> Mux_AutomatedDrivingFunction_ACC/7  "<Key_1_Idx[]>"
  Bus_Selector_AutomatedDrivingFunction_ACC/8 -> Mux_AutomatedDrivingFunction_ACC/8  "<Value_1_Idx[]>"
  Bus_Selector_AutomatedDrivingFunction_ACC/9 -> Mux_AutomatedDrivingFunction_ACC/9  "<Key_2_Idx[]>"
  Bus_Selector_AutomatedDrivingFunction_ACC/10 -> Mux_AutomatedDrivingFunction_ACC/10  "<Value_2_Idx[]>"
  Bus_Selector_AutomatedDrivingFunction_AEB/1 -> Mux_AutomatedDrivingFunction_AEB/1  "<Driver_Override_Reason_Idx[]>"
  Bus_Selector_AutomatedDrivingFunction_AEB/2 -> Mux_AutomatedDrivingFunction_AEB/2  "<Driver_Override_Reason_Idx[]>"
  Bus_Selector_AutomatedDrivingFunction_AEB/3 -> Mux_AutomatedDrivingFunction_AEB/3  "<State_Idx[]>"
  Bus_Selector_AutomatedDrivingFunction_AEB/4 -> Mux_AutomatedDrivingFunction_AEB/4  "<Name_Idx[]>"
  Bus_Selector_AutomatedDrivingFunction_AEB/5 -> Mux_AutomatedDrivingFunction_AEB/5  "<Custom_Name_Idx[]>"
  Bus_Selector_AutomatedDrivingFunction_AEB/6 -> Mux_AutomatedDrivingFunction_AEB/6  "<Custom_State_Idx[]>"
  Bus_Selector_AutomatedDrivingFunction_AEB/7 -> Mux_AutomatedDrivingFunction_AEB/7  "<Key_1_Idx[]>"
  Bus_Selector_AutomatedDrivingFunction_AEB/8 -> Mux_AutomatedDrivingFunction_AEB/8  "<Value_1_Idx[]>"
  Bus_Selector_AutomatedDrivingFunction_AEB/9 -> Mux_AutomatedDrivingFunction_AEB/9  "<Key_2_Idx[]>"
  Bus_Selector_AutomatedDrivingFunction_AEB/10 -> Mux_AutomatedDrivingFunction_AEB/10  "<Value_2_Idx[]>"
  Bus_Selector_AutomatedDrivingFunction_FCW/1 -> Mux_AutomatedDrivingFunction_FCW/1  "<Driver_Override_Active[0Off|1On]>"
  Bus_Selector_AutomatedDrivingFunction_FCW/2 -> Mux_AutomatedDrivingFunction_FCW/2  "<Driver_Override_Reason_Idx[]>"
  Bus_Selector_AutomatedDrivingFunction_FCW/3 -> Mux_AutomatedDrivingFunction_FCW/3  "<State_Idx[]>"
  Bus_Selector_AutomatedDrivingFunction_FCW/4 -> Mux_AutomatedDrivingFunction_FCW/4  "<Name_Idx[]>"
  Bus_Selector_AutomatedDrivingFunction_FCW/5 -> Mux_AutomatedDrivingFunction_FCW/5  "<Custom_Name_Idx[]>"
  Bus_Selector_AutomatedDrivingFunction_FCW/6 -> Mux_AutomatedDrivingFunction_FCW/6  "<Custom_State_Idx[]>"
  Bus_Selector_AutomatedDrivingFunction_FCW/7 -> Mux_AutomatedDrivingFunction_FCW/7  "<Key_1_Idx[]>"
  Bus_Selector_AutomatedDrivingFunction_FCW/8 -> Mux_AutomatedDrivingFunction_FCW/8  "<Value_1_Idx[]>"
  Bus_Selector_AutomatedDrivingFunction_FCW/9 -> Mux_AutomatedDrivingFunction_FCW/9  "<Key_2_Idx[]>"
  Bus_Selector_AutomatedDrivingFunction_FCW/10 -> Mux_AutomatedDrivingFunction_FCW/10  "<Value_2_Idx[]>"
  Bus_Selector_AutomatedDrivingFunction_4/1 -> Mux_AutomatedDrivingFunction_4/1  "<Driver_Override_Active[0Off|1On]>"
  Bus_Selector_AutomatedDrivingFunction_4/2 -> Mux_AutomatedDrivingFunction_4/2  "<Driver_Override_Reason_Idx[]>"
  Bus_Selector_AutomatedDrivingFunction_4/3 -> Mux_AutomatedDrivingFunction_4/3  "<State_Idx[]>"
  Bus_Selector_AutomatedDrivingFunction_4/4 -> Mux_AutomatedDrivingFunction_4/4  "<Name_Idx[]>"
  Bus_Selector_AutomatedDrivingFunction_4/5 -> Mux_AutomatedDrivingFunction_4/5  "<Custom_Name_Idx[]>"
  Bus_Selector_AutomatedDrivingFunction_4/6 -> Mux_AutomatedDrivingFunction_4/6  "<Custom_State_Idx[]>"
  Bus_Selector_AutomatedDrivingFunction_4/7 -> Mux_AutomatedDrivingFunction_4/7  "<Key_1_Idx[]>"
  Bus_Selector_AutomatedDrivingFunction_4/8 -> Mux_AutomatedDrivingFunction_4/8  "<Value_1_Idx[]>"
  Bus_Selector_AutomatedDrivingFunction_4/9 -> Mux_AutomatedDrivingFunction_4/9  "<Key_2_Idx[]>"
  Bus_Selector_AutomatedDrivingFunction_4/10 -> Mux_AutomatedDrivingFunction_4/10  "<Value_2_Idx[]>"
  Mux_AutomatedDrivingFunction_ACC/1 -> Mux4/1
  Mux_AutomatedDrivingFunction_AEB/1 -> Mux4/2
  Mux_AutomatedDrivingFunction_FCW/1 -> Mux4/3
  Mux_AutomatedDrivingFunction_4/1 -> Mux4/4
  Mux4/1 -> AutomatedDrivingFunction[]/1

== system ASM_Traffic_MultiCore/Environment/GroundTruth/PlantModel/GetFellowPositionVector ==
  FellowPositions : Inport
  Bus Selector11 : BusSelector  OutputSignals=Pos_Fellows_MainPnt_CoorSys_E[x;y;z][m].Pos_x_Fellows[m],Pos_Fellows_MainPnt_CoorSys_E[x;y;z][m].Pos_y_Fellows[m],Pos_Fellows_MainPnt_CoorSys_E[x;y;z][m].Pos_z_Fellows[m],Angle_Fellows[x;y;z][deg].Angle_Roll_Fellows[deg],Angle_Fellows[x;y;z][deg].Angle_Pitch_Fellows[deg],Angle_Fellows[x;y;z][deg].Angle_Yaw_Fellows[deg]
  Mux1 : Mux  Inputs=3
  Mux2 : Mux  Inputs=3
  Pos_Fellows_MainPnt_CoorSys_E[x;y;z][m] : Outport  VectorParamsAs1DForOutWhenUnconnected=off
  Angle_Fellows[deg] : Outport  Port=2  VectorParamsAs1DForOutWhenUnconnected=off
  wires:
  Mux2/1 -> Pos_Fellows_MainPnt_CoorSys_E[x;y;z][m]/1  "Pos_Fellows_MainPnt_CoorSys_E[x;y;z][m]"
  Mux1/1 -> Angle_Fellows[deg]/1  "Pos_Fellows_MainPnt_CoorSys_E_vec"
  Bus Selector11/4 -> Mux1/1  "<Angle_Roll_Fellows[deg]>"
  Bus Selector11/1 -> Mux2/1  "<Pos_x_Fellows[m]>"
  Bus Selector11/2 -> Mux2/2  "<Pos_y_Fellows[m]>"
  Bus Selector11/6 -> Mux1/3  "<Angle_Yaw_Fellows[deg]>"
  Bus Selector11/5 -> Mux1/2  "<Angle_Pitch_Fellows[deg]>"
  FellowPositions/1 -> Bus Selector11/1
  Bus Selector11/3 -> Mux2/3  "<Pos_z_Fellows[m]>"
